simulink library "lib_AC_GFL"  (R2026a)
settings: Solver=VariableStepAuto
undefined symbols (not defined in the file): block_buses, block_idx, block_toM, buses_lf, CCVSC_idx, fref, invL, iPs_lf, iQs_lf, iTf, op_GFL
libraries: sl_discontinuities x2
settings Model: Creator=atomas  LastModifiedBy=atomas

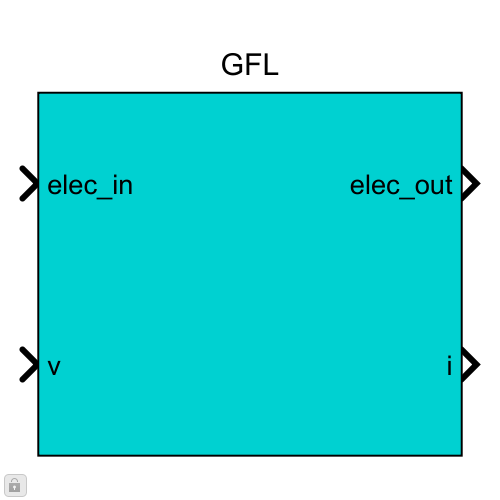
[thumbnail: Simulink's stored preview of the top-level diagram]
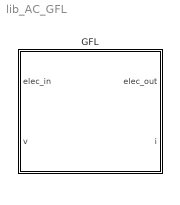
== system lib_AC_GFL ==
  GFL : Subsystem  mask(GFl){Pmax=0, Qmax=0, fb=50, dynamic_CC=Static, Tint=0.1, Kint=1, Bint=1, Lf=0.01, Rf=0.001, dynamic_PLL=Dynamic, kpi=1, kii=10, Tf=0, alphapcoef=0, alphaqcoef=0, Prel=1, Qrel=1, Eref=1}
      mask prompts: Pmax "Active power limit (p.u.)"; Qmax "Reactive power limit (p.u.)"; fb "Base frequency (Hz)"; dynamic_CC "Dynamic behaviour"; Lf "Filter inductance"; Rf "Filter resistance"; dynamic_PLL "Dynamic behaviour"; Tf "LPF time constant (s)"; alphapcoef "P droop coefficient"; alphaqcoef "Q droop coefficient"; Prel "P/P_NmP"; Qrel "Q/Q_NnQ"; Eref "Nominal voltage of PCC"
      mask help: Grid-following converter. CC is the current controller. Dynamic behavior includes the PI controller, decoupling and output inductance. Static behavior consists of setting the reference current directly in the output. PC is the power controller including the current reference calculation and low-pass filters for the power measurements.
      mask init:
      | [block_buses, block_idx, block_toM, block_fref, iTf, use_Tf, cc_mode, pll_mode] = mask_init_GFL(gcb, Tf, dynamic_CC, dynamic_PLL);
      mask Help: web('doc_GFl.html')
      mask TypeOptions dynamic_CC: Dynamic | Static
      mask TypeOptions dynamic_PLL: Dynamic | Static
      mask DialogControl CC Prompt: CC
      mask DialogControl PLL Prompt: PLL
      mask DialogControl PC Prompt: PC

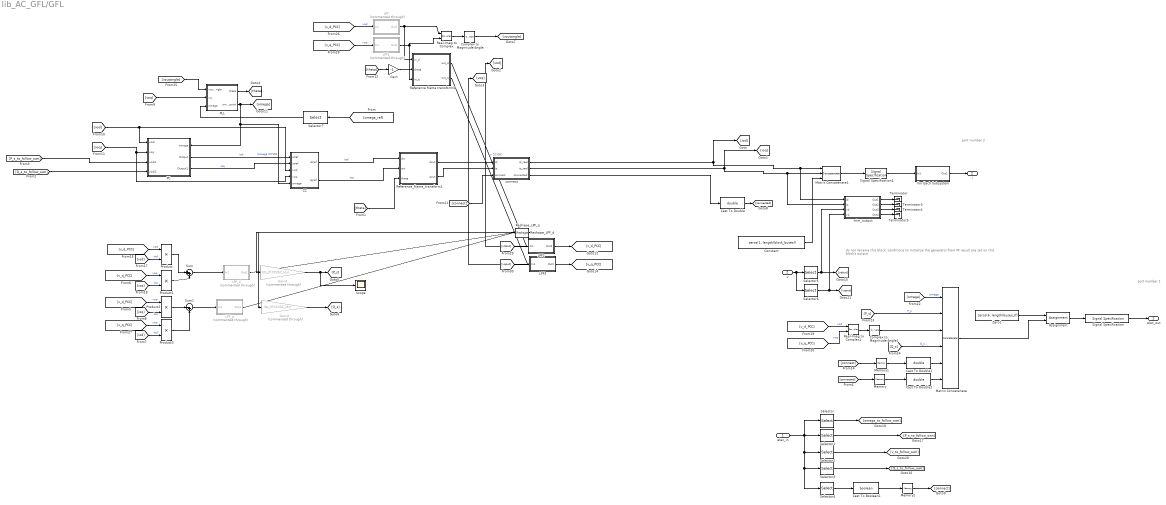
== system lib_AC_GFL/GFL ==
  note: do not rename this block, conditions to initialise the generator from PF result are set on this block's output
  note: port number 1
  note: port number 2
  elec_in : Inport
  v : Inport  Port=2
  Assignment : Assignment  NumberOfDimensions=2  DiagnosticForDimensions=Warning  IndexOptions=Assign all,Index vector (dialog)  Indices=1,block_idx  OutputSizes=1,1
  CC : Subsystem  Variant=on
  Cast To Boolean1 : DataTypeConversion  OutDataTypeStr=boolean  SaturateOnIntegerOverflow=off  RndMeth=Floor
  Cast To Double : DataTypeConversion  OutDataTypeStr=double  SaturateOnIntegerOverflow=off  RndMeth=Floor
  Cast To Double1 : DataTypeConversion  OutDataTypeStr=double  SaturateOnIntegerOverflow=off  RndMeth=Floor
  Cast To Double2 : DataTypeConversion  OutDataTypeStr=double  SaturateOnIntegerOverflow=off  RndMeth=Floor
  Complex to Magnitude-Angle : ComplexToMagnitudeAngle  Output=Angle
  Complex to Magnitude-Angle1 : ComplexToMagnitudeAngle  Output=Magnitude
  Constant : Constant  Value=zeros(1, length(block_buses))  VectorParams1D=off
  For Each Subsystem : Subsystem  TreatAsAtomicUnit=on
  Gain : Gain  Gain=-1
  Gain3 : Gain  Commented=through  Gain=iQs_lf(CCVSC_idx)
  Gain4 : Gain  Commented=through  Gain=iPs_lf(CCVSC_idx)
  LPF : Subsystem  Commented=through
  LPF1 : Subsystem  Commented=through
  LPF2 : Subsystem
  LPF3 : Subsystem
  LPF_d : Subsystem  Commented=through  Variant=on
  LPF_q : Subsystem  Commented=through  Variant=on
  Matrix Concatenate : Concatenate  NumInputs=6  Mode=Multidimensional array
  Matrix Concatenate1 : Concatenate  NumInputs=3  Mode=Multidimensional array
  Memory : Memory  InitialCondition=1
  Memory1 : Memory  InitialCondition=1
  Memory2 : Memory  InitialCondition=1
  PC : Subsystem
      settings: PortSchema="{\"entries\":[{\"content\":{\"sides\":[{\"content\":{\"connectorIds\":[\"In1\",\"In2\",\"In3\",\"In4\"]},\"type\":\"ConnectorPlacement.EquallySpacedRectSide\",\"uuid\":\"7748ce6f-2dcc-431c-b3ea-0be9c3088b1d\"},{\"content\":{\"connectorIds\":[\"In5\",\"Out1\",\"Out2\"],\"side\":\"RIGHT\"},\"type\":\"ConnectorPlacement.EquallySpacedRectSide\",\"uuid\":\"af86fd8d-043b-4d20-8ee8-e7a977d706a8\"},{\"content\":{\"connectorIds\":[],\"side\":\"TOP\"},\"type\":\"ConnectorPlacement.EquallySpacedRectSide\",\"uuid\":\"807e0dc6-0d59-4ea5-9557-3ccfd29c2ad0\"}]},\"type\":\"ConnectorPlacement.EquallySpacedConnector\",\"uuid\":\"c7fe00c5-0a0a-4038-b7ac-e659fb2aa4a7\"}],\"packageUris\":[\"http://schema.mathworks.com/mf0/Connector/R2020b\"],\"version\":\"1.0\"}"
  PLL : Subsystem  Variant=on
  Product{,1..3} (4 alike) : Product
  Real-Imag to Complex : RealImagToComplex
  Real-Imag to Complex1 : RealImagToComplex
  Reference frame transform3 : Subsystem
  Reference_frame_transform1 : Subsystem
  Reshape_LPF_d : Reshape  OutputDimensionality=Row vector (2-D)
  Reshape_LPF_q : Reshape  OutputDimensionality=Row vector (2-D)
  Scope : Scope
      settings: DataLoggingVariableName=ScopeData8
  Selector : Selector  NumberOfDimensions=2  InputPortWidth=3  IndexOptions=Index vector (dialog),Index vector (dialog)  Indices=1,block_idx  OutputSizes=1,1
  Selector1 : Selector  NumberOfDimensions=2  InputPortWidth=3  IndexOptions=Index vector (dialog),Index vector (dialog)  Indices=2,block_idx  OutputSizes=1,1
  Selector2 : Selector  NumberOfDimensions=2  InputPortWidth=3  IndexOptions=Index vector (dialog),Index vector (dialog)  Indices=3,block_idx  OutputSizes=1,1
  Selector3 : Selector  NumberOfDimensions=2  InputPortWidth=3  IndexOptions=Index vector (dialog),Index vector (dialog)  Indices=4,block_idx  OutputSizes=1,1
  Selector4 : Selector  NumberOfDimensions=2  InputPortWidth=3  IndexOptions=Index vector (dialog),Index vector (dialog)  Indices=5,block_idx  OutputSizes=1,1
  Selector5 : Selector  NumberOfDimensions=2  InputPortWidth=3  IndexOptions=Index vector (dialog),Index vector (dialog)  Indices=1,block_buses  OutputSizes=1,1
  Selector6 : Selector  NumberOfDimensions=2  InputPortWidth=3  IndexOptions=Index vector (dialog),Index vector (dialog)  Indices=2,block_buses  OutputSizes=1,1
  Selector7 : Selector  InputPortWidth=length(fref.ref_units)  IndexOptions=Index vector (dialog)  Indices=block_fref  OutputSizes=1
  Signal Specification : SignalSpecification  Dimensions=[6 length(buses_lf)]
  Signal Specification1 : SignalSpecification  Dimensions=[3 length(block_buses)]
  Sum : Sum  Inputs=|++
  Sum1 : Sum  Inputs=|-+
  Terminator{,3..5} (4 alike) : Terminator
  Zero1 : Constant  Value=zeros(6, length(buses_lf))  VectorParams1D=off  OutDataTypeStr=Inherit: Inherit via back propagation
  connect : Subsystem
  trim_output : Subsystem
  elec_out : Outport
  i : Outport  Port=2
  wires:
  Sum1/1 -> LPF_q/1(In1)
  Sum/1 -> LPF_d/1(In1)
  [voutangle] -> PLL/1(voutangle)
  [Q_s_to_follow_own] -> PC/4(vodi2)
  [P_s_to_follow_own] -> PC/3(vodi1)
  connect/3(connected) -> Cast To Double/1
  CC/2(iqiref) -> Reference_frame_transform1/2(qin)  "ioq"
  CC/1(idiref) -> Reference_frame_transform1/1(din)  "iod"
  PLL/1(theta) -> [theta]
  [omega_ref] -> Selector7/1
  [voq] -> PLL/2(vq)
  [theta] -> Reference_frame_transform1/3(theta)
  Gain/1 -> Reference frame transform3/2(theta)
  [theta] -> Gain/1
  PC/2(Output1) -> CC/2(iqref)  "ioq"
  PC/1(Output) -> CC/1(idref)  "iod"
  [v_q_PCC] -> Product3/1  "voq"
  [v_d_PCC] -> Product2/1  "vod"
  [ioq] -> Product1/2  "ioq"
  [iod] -> Product/2  "iod"
  [v_d_PCC] -> Product/1  "vod"
  Gain3/1 -> [Q_s]
  Gain4/1 -> Scope/1, [P_s]
  Product/1 -> Sum/1
  Product3/1 -> Sum1/2
  Product1/1 -> Sum/2
  Product2/1 -> Sum1/1
  [ioq] -> Product2/2  "ioq"
  [iod] -> Product3/2  "iod"
  [v_q_PCC] -> Product1/1  "voq"
  [voq] -> PC/2(voq), CC/4(voq)
  [vod] -> PC/1(vodi), CC/3(vod)
  Real-Imag to Complex/1 -> Complex to Magnitude-Angle/1
  Complex to Magnitude-Angle/1 -> [voutangle]
  PLL/2(omega_point) -> PC/5(omega), CC/5(omega), [omega]  "\\omega CCVSC"
  Reference_frame_transform1/2(qout) -> connect/2(iq)
  Reference_frame_transform1/1(dout) -> connect/1(id)
  Selector3/1 -> [Q_s_to_follow_own]
  Selector2/1 -> [v_to_follow_own]
  Selector/1 -> [omega_to_follow_own]
  [omega] -> Matrix Concatenate/1  "omega"
  [P_s] -> Matrix Concatenate/2  "P_s"
  [Q_s] -> Matrix Concatenate/4  "Q_s"
  [connected] -> Memory/1
  [connect] -> Memory1/1
  Cast To Double/1 -> [connected]
  [connect] -> connect/3(connect)
  connect/1(id_real) -> [iod], trim_output/1(id), Matrix Concatenate1/1
  connect/2(iq_real) -> [ioq], trim_output/2(iq), Matrix Concatenate1/2
  [v_d_PCC] -> Real-Imag to Complex1/1  "vod"
  [v_q_PCC] -> Real-Imag to Complex1/2  "voq"
  Real-Imag to Complex1/1 -> Complex to Magnitude-Angle1/1
  Complex to Magnitude-Angle1/1 -> Matrix Concatenate/3
  [v_d_PCC] -> LPF/1(In1)  "vod"
  [v_q_PCC] -> LPF1/1(In1)  "voq"
  Selector4/1 -> Cast To Boolean1/1
  Cast To Boolean1/1 -> Memory2/1
  Cast To Double1/1 -> Matrix Concatenate/5
  Cast To Double2/1 -> Matrix Concatenate/6
  Zero1/1 -> Assignment/1
  Signal Specification/1 -> elec_out/1
  Assignment/1 -> Signal Specification/1
  Matrix Concatenate/1 -> Assignment/2
  elec_in/1 -> Selector4/1, Selector3/1, Selector2/1, Selector1/1, Selector/1
  Matrix Concatenate1/1 -> Signal Specification1/1
  Signal Specification1/1 -> For Each Subsystem/1(In1)
  Constant/1 -> Matrix Concatenate1/3
  For Each Subsystem/1(Out1) -> i/1
  trim_output/1(Out1) -> Terminator/1
  trim_output/3(Out3) -> Terminator4/1
  trim_output/2(Out2) -> Terminator3/1
  trim_output/4(Out4) -> Terminator5/1
  Selector5/1 -> trim_output/3(vd), [vdout]
  Selector6/1 -> trim_output/4(vq), [vqout]
  v/1 -> Selector6/1, Selector5/1
  Memory/1 -> Cast To Double2/1
  Selector1/1 -> [P_s_to_follow_own]
  Memory1/1 -> Cast To Double1/1
  Memory2/1 -> [connect]
  LPF/1(Out1) -> Reference frame transform3/1(in_d), Real-Imag to Complex/1
  LPF1/1(Out1) -> Real-Imag to Complex/2, Reference frame transform3/3(in_q)
  Selector7/1 -> PLL/3(omega)
  [vdout] -> [v_d_PCC]
  [vqout] -> [v_q_PCC]
  Reference frame transform3/1(out_d) -> LPF2/1(In1)  "v CCVSC"
  LPF2/1(Out1) -> [vod]
  Reference frame transform3/2(out_q) -> LPF3/1(In1)
  LPF3/1(Out1) -> [voq]
  LPF_d/1(Out1) -> Reshape_LPF_d/1
  Reshape_LPF_d/1 -> Gain4/1
  LPF_q/1(Out1) -> Reshape_LPF_q/1
  Reshape_LPF_q/1 -> Gain3/1

== system lib_AC_GFL/GFL/CC ==
  note: 1) Add Subsystem or Model blocks as valid variant choices.
      | 2) You cannot connect blocks at this level. At simulation, connectivity is automatically
      | determined, based on the active variant and port name matching.
  idref : Inport
  iqref : Inport  Port=2
  vod : Inport  Port=3
  voq : Inport  Port=4
  omega : Inport  Port=5
  dynamic : Subsystem  VariantControl=cc_mode == 1  mask{dynamic_line=Dynamic}
      mask prompts: dynamic_line "Line"
      mask TypeOptions dynamic_line: RL/dynamic
  static : Subsystem  VariantControl=(default)
  idiref : Outport
  iqiref : Outport  Port=2

== system lib_AC_GFL/GFL/For Each Subsystem ==
  In1 : Inport  Partition=on  PartitionDimension=1  PartitionWidth=1  PartitionOffset=0
  For Each : ForEach  DisableCoverage=on
  State-Space : StateSpace  A=[]  B=[]  C=[]  D=block_toM  InitialCondition=0  ParameterTunability=Optimized
  Transpose : Math  Operator=transpose
  Transpose1 : Math  Operator=transpose
  Out1 : Outport  ConcatenationDimension=1
  wires:
  Transpose1/1 -> Out1/1
  In1/1 -> Transpose/1
  Transpose/1 -> State-Space/1
  State-Space/1 -> Transpose1/1

== system lib_AC_GFL/GFL/LPF ==
  In1 : Inport
  Gain : Gain  Gain=1e2
  I : Integrator  InitialCondition=op_GFL.LPF_I
  Sum4 : Sum  Inputs=|+-
  Out1 : Outport
  wires:
  Gain/1 -> I/1
  Sum4/1 -> Gain/1
  In1/1 -> Sum4/1
  I/1 -> Out1/1, Sum4/2

== system lib_AC_GFL/GFL/LPF1 ==
  In1 : Inport
  Gain : Gain  Gain=1e2
  I : Integrator  InitialCondition=op_GFL.LPF1_I
  Sum4 : Sum  Inputs=|+-
  Out1 : Outport
  wires:
  I/1 -> Sum4/2, Out1/1
  In1/1 -> Sum4/1
  Sum4/1 -> Gain/1
  Gain/1 -> I/1

== system lib_AC_GFL/GFL/LPF2 ==
  In1 : Inport
  Gain : Gain  Gain=1e2
  I : Integrator  InitialCondition=op_GFL.LPF2_I
  Sum4 : Sum  Inputs=|+-
  Out1 : Outport
  wires:
  Gain/1 -> I/1
  Sum4/1 -> Gain/1
  In1/1 -> Sum4/1
  I/1 -> Out1/1, Sum4/2

== system lib_AC_GFL/GFL/LPF3 ==
  In1 : Inport
  Gain : Gain  Gain=1e2
  I : Integrator  InitialCondition=op_GFL.LPF3_I
  Sum4 : Sum  Inputs=|+-
  Out1 : Outport
  wires:
  I/1 -> Sum4/2, Out1/1
  In1/1 -> Sum4/1
  Sum4/1 -> Gain/1
  Gain/1 -> I/1

== system lib_AC_GFL/GFL/LPF_d ==
  note: 1) Add Subsystem or Model blocks as valid variant choices.
      | 2) You cannot connect blocks at this level. At simulation, connectivity is automatically
      | determined, based on the active variant and port name matching.
  In1 : Inport
  Active : Subsystem  VariantControl=use_Tf == 1
  Bypass : Subsystem  VariantControl=(default)
  Out1 : Outport

== system lib_AC_GFL/GFL/LPF_q ==
  note: 1) Add Subsystem or Model blocks as valid variant choices.
      | 2) You cannot connect blocks at this level. At simulation, connectivity is automatically
      | determined, based on the active variant and port name matching.
  In1 : Inport
  Active : Subsystem  VariantControl=use_Tf == 1
  Bypass : Subsystem  VariantControl=(default)
  Out1 : Outport

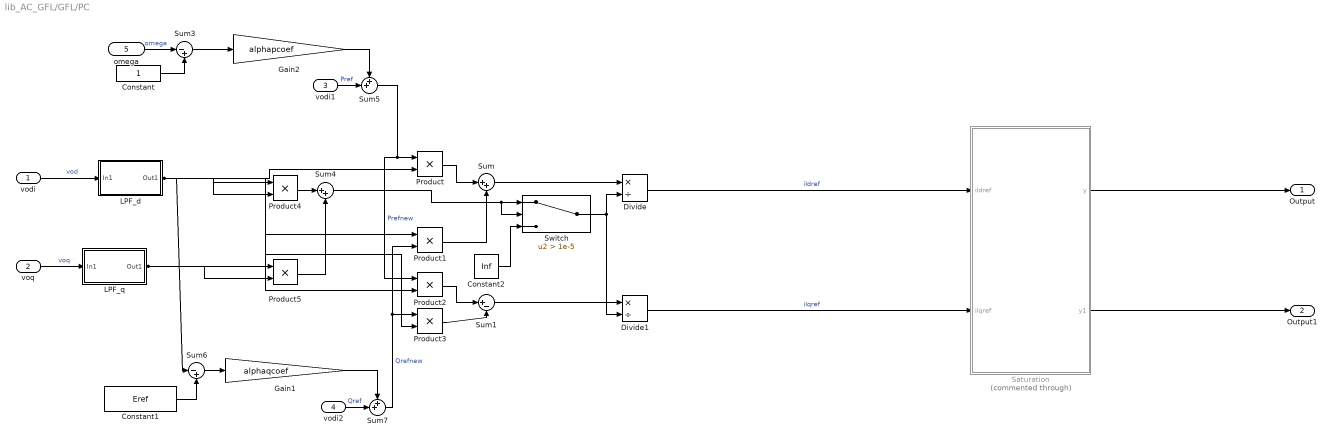
== system lib_AC_GFL/GFL/PC ==
  vodi : Inport
  voq : Inport  Port=2
  vodi1 : Inport  Port=3
  vodi2 : Inport  Port=4
  omega : Inport  Port=5
  Constant : Constant
  Constant1 : Constant  Value=Eref  VectorParams1D=off
  Constant2 : Constant  Value=Inf
  Divide : Product  Inputs=*/
  Divide1 : Product  Inputs=*/
  Gain1 : Gain  Gain=alphaqcoef
  Gain2 : Gain  Gain=alphapcoef
  LPF_d : Subsystem  Variant=on
  LPF_q : Subsystem  Variant=on
  Product{,1..5} (6 alike) : Product
  Saturation : Subsystem  Commented=through
  Sum : Sum  Inputs=|++
  Sum1 : Sum  Inputs=|+-
  Sum3 : Sum  Inputs=|-+
  Sum4 : Sum  Inputs=|++
  Sum5 : Sum  Inputs=++|
  Sum6 : Sum  Inputs=|-+
  Sum7 : Sum  Inputs=++|
  Switch : Switch  Criteria=u2 > Threshold  Threshold=1e-5  ZeroCross=off  SaturateOnIntegerOverflow=off  InputSameDT=off
  Output : Outport
  Output1 : Outport  Port=2
  wires:
  LPF_q/1(Out1) -> Product5/1, Product5/2, Product2/2, Product1/1
  voq/1 -> LPF_q/1(In1)  "voq"
  LPF_d/1(Out1) -> Product4/1, Product4/2, Product/2, Product3/2, Sum6/1
  vodi/1 -> LPF_d/1(In1)  "vod"
  Switch/1 -> Divide1/2, Divide/2
  Constant2/1 -> Switch/3
  vodi2/1 -> Sum7/2  "Qref"
  Sum6/1 -> Gain1/1
  omega/1 -> Sum3/1  "omega"
  Gain1/1 -> Sum7/1
  Constant1/1 -> Sum6/2
  vodi1/1 -> Sum5/2  "Pref"
  Gain2/1 -> Sum5/1
  Constant/1 -> Sum3/2
  Sum3/1 -> Gain2/1
  Sum/1 -> Divide/1
  Sum4/1 -> Switch/1, Switch/2
  Sum1/1 -> Divide1/1
  Sum5/1 -> Product/1, Product2/1  "Prefnew"
  Product5/1 -> Sum4/2
  Product4/1 -> Sum4/1
  Sum7/1 -> Product3/1, Product1/2  "Qrefnew"
  Product3/1 -> Sum1/2
  Product2/1 -> Sum1/1
  Product1/1 -> Sum/2
  Product/1 -> Sum/1
  Divide/1 -> Saturation/1(ildref)  "ildref"
  Divide1/1 -> Saturation/2(ilqref)  "ilqref"
  Saturation/1(y) -> Output/1
  Saturation/2(y1) -> Output1/1

== system lib_AC_GFL/GFL/PLL ==
  note: 1) Add Subsystem or Model blocks as valid variant choices.
      | 2) You cannot connect blocks at this level. At simulation, connectivity is automatically
      | determined, based on the active variant and port name matching.
  voutangle : Inport
  vq : Inport  Port=2
  omega : Inport  Port=3
  dynamic : Subsystem  VariantControl=pll_mode == 1
  static : Subsystem  VariantControl=(default)
  theta : Outport
  omega_point : Outport  Port=2

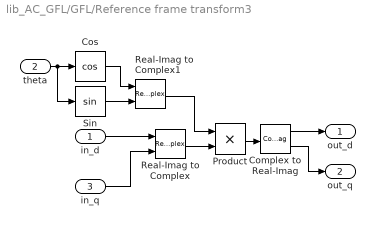
== system lib_AC_GFL/GFL/Reference frame transform3 ==
  in_d : Inport
  theta : Inport  Port=2
  in_q : Inport  Port=3
  Complex to Real-Imag : ComplexToRealImag
  Cos : Trigonometry  SCDEnableBlockLinearizationSpecification=on  Operator=cos
  Product : Product
  Real-Imag to Complex : RealImagToComplex
  Real-Imag to Complex1 : RealImagToComplex
  Sin : Trigonometry  SCDEnableBlockLinearizationSpecification=on
  out_d : Outport
  out_q : Outport  Port=2
  wires:
  Complex to Real-Imag/2 -> out_q/1
  Real-Imag to Complex1/1 -> Product/1
  Real-Imag to Complex/1 -> Product/2
  Product/1 -> Complex to Real-Imag/1
  theta/1 -> Sin/1, Cos/1
  Cos/1 -> Real-Imag to Complex1/1
  Sin/1 -> Real-Imag to Complex1/2
  Complex to Real-Imag/1 -> out_d/1
  in_q/1 -> Real-Imag to Complex/2
  in_d/1 -> Real-Imag to Complex/1

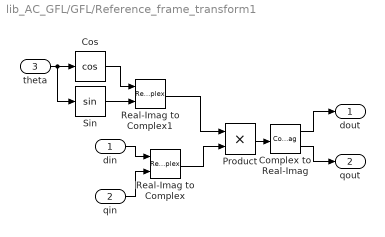
== system lib_AC_GFL/GFL/Reference_frame_transform1 ==
  din : Inport
  qin : Inport  Port=2
  theta : Inport  Port=3
  Complex to Real-Imag : ComplexToRealImag
  Cos : Trigonometry  SCDEnableBlockLinearizationSpecification=on  Operator=cos
  Product : Product
  Real-Imag to Complex : RealImagToComplex
  Real-Imag to Complex1 : RealImagToComplex
  Sin : Trigonometry  SCDEnableBlockLinearizationSpecification=on
  dout : Outport
  qout : Outport  Port=2
  wires:
  Sin/1 -> Real-Imag to Complex1/2
  Cos/1 -> Real-Imag to Complex1/1
  theta/1 -> Cos/1, Sin/1
  Product/1 -> Complex to Real-Imag/1
  Real-Imag to Complex/1 -> Product/2
  qin/1 -> Real-Imag to Complex/2
  din/1 -> Real-Imag to Complex/1
  Real-Imag to Complex1/1 -> Product/1
  Complex to Real-Imag/2 -> qout/1
  Complex to Real-Imag/1 -> dout/1

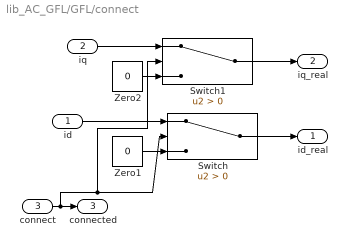
== system lib_AC_GFL/GFL/connect ==
  id : Inport
  iq : Inport  Port=2
  connect : Inport  Port=3
  Switch : Switch  Criteria=u2 > Threshold  ZeroCross=off  SaturateOnIntegerOverflow=off  InputSameDT=off
  Switch1 : Switch  Criteria=u2 > Threshold  ZeroCross=off  SaturateOnIntegerOverflow=off  InputSameDT=off
  Zero1 : Constant  Value=0  VectorParams1D=off  OutDataTypeStr=Inherit: Inherit via back propagation
  Zero2 : Constant  Value=0  VectorParams1D=off  OutDataTypeStr=Inherit: Inherit via back propagation
  id_real : Outport
  iq_real : Outport  Port=2
  connected : Outport  Port=3  OutDataTypeStr=boolean
  wires:
  Switch/1 -> id_real/1
  Zero1/1 -> Switch/3
  id/1 -> Switch/1
  connect/1 -> connected/1, Switch1/2, Switch/2
  Switch1/1 -> iq_real/1
  iq/1 -> Switch1/1
  Zero2/1 -> Switch1/3

== system lib_AC_GFL/GFL/trim_output ==
  id : Inport
  iq : Inport  Port=2
  vd : Inport  Port=3
  vq : Inport  Port=4
  Out1 : Outport
  Out2 : Outport  Port=2
  Out3 : Outport  Port=3
  Out4 : Outport  Port=4
  wires:
  id/1 -> Out1/1
  vq/1 -> Out4/1
  vd/1 -> Out3/1
  iq/1 -> Out2/1

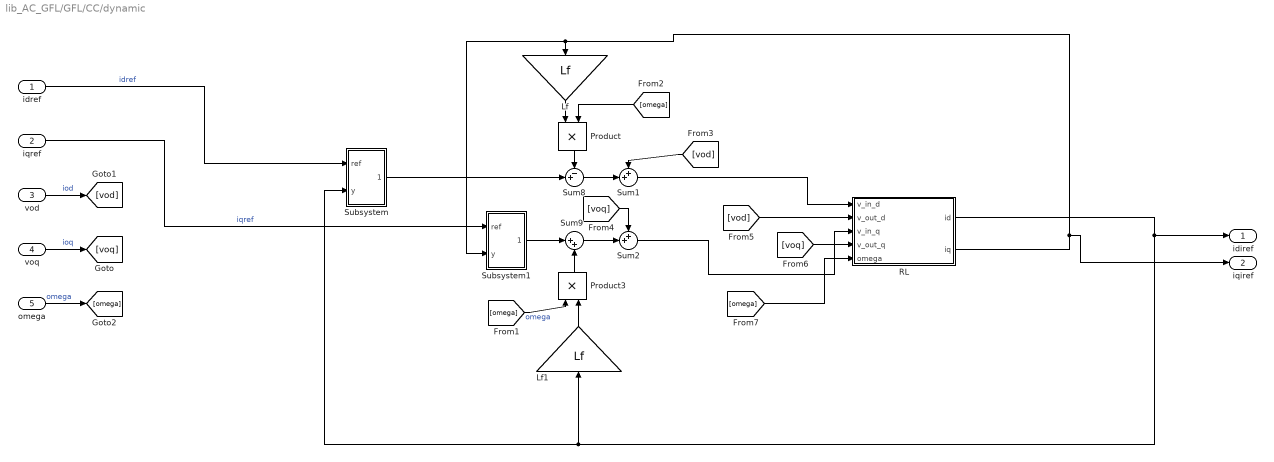
== system lib_AC_GFL/GFL/CC/dynamic ==
  idref : Inport
  iqref : Inport  Port=2
  vod : Inport  Port=3
  voq : Inport  Port=4
  omega : Inport  Port=5
  "Lf " : Gain  Gain=Lf
  Lf1 : Gain  Gain=Lf
  Product : Product
  Product3 : Product
  RL : Subsystem  Variant=on  mask(Line){dynamic=Dynamic, R=Rf, L=Lf}
      mask prompts: dynamic "Dynamic behavior"; R "Series resistance (p.u.)"; L "Inductance (p.u.)"
      mask init:
      | [invL, omegab, rl_mode] = mask_init_RL(dynamic, L, 50);
      mask Help: web('Documentation/RL.html')
      mask TypeOptions dynamic: Static | Dynamic | Static omega
  Subsystem : Subsystem
  Subsystem1 : Subsystem
  Sum1 : Sum  Inputs=++|
  Sum2 : Sum  Inputs=++|
  Sum8 : Sum  Inputs=-+|
  Sum9 : Sum  Inputs=|++
  idiref : Outport
  iqiref : Outport  Port=2
  wires:
  RL/2(iq) -> iqiref/1, Subsystem1/2(y), "Lf "/1
  Subsystem1/1(Out1) -> Sum9/1
  [omega] -> Product3/1  "omega"
  "Lf "/1 -> Product/1
  Product3/1 -> Sum9/2
  Lf1/1 -> Product3/2
  [omega] -> Product/2
  Product/1 -> Sum8/1
  iqref/1 -> Subsystem1/1(ref)  "iqref"
  Sum8/1 -> Sum1/2
  Sum9/1 -> Sum2/2
  [vod] -> Sum1/1
  [voq] -> Sum2/1
  omega/1 -> [omega]  "omega"
  voq/1 -> [voq]  "ioq"
  vod/1 -> [vod]  "iod"
  [vod] -> RL/2(v_out_d)
  [voq] -> RL/4(v_out_q)
  Sum1/1 -> RL/1(v_in_d)
  Sum2/1 -> RL/3(v_in_q)
  RL/1(id) -> Subsystem/2(y), Lf1/1, idiref/1
  idref/1 -> Subsystem/1(ref)  "idref"
  Subsystem/1(Out1) -> Sum8/2
  [omega] -> RL/5(omega)

== system lib_AC_GFL/GFL/CC/static ==
  idref : Inport
  iqref : Inport  Port=2
  vod : Inport  Port=3
  voq : Inport  Port=4
  omega : Inport  Port=5
  Terminator : Terminator
  Terminator1 : Terminator
  Terminator2 : Terminator
  idiref : Outport
  iqiref : Outport  Port=2
  wires:
  voq/1 -> Terminator1/1  "voq"
  vod/1 -> Terminator/1  "vod"
  idref/1 -> idiref/1  "idref"
  iqref/1 -> iqiref/1  "iqref"
  omega/1 -> Terminator2/1  "omega"

== system lib_AC_GFL/GFL/LPF_d/Active ==
  In1 : Inport
  Impl : Subsystem
  Out1 : Outport
  wires:
  Impl/1(Out1) -> Out1/1
  In1/1 -> Impl/1(In1)

== system lib_AC_GFL/GFL/LPF_d/Bypass ==
  In1 : Inport
  Reshape_row : Reshape  OutputDimensionality=Row vector (2-D)
  Out1 : Outport
  wires:
  In1/1 -> Reshape_row/1
  Reshape_row/1 -> Out1/1

== system lib_AC_GFL/GFL/LPF_q/Active ==
  In1 : Inport
  Impl : Subsystem
  Out1 : Outport
  wires:
  Impl/1(Out1) -> Out1/1
  In1/1 -> Impl/1(In1)

== system lib_AC_GFL/GFL/LPF_q/Bypass ==
  In1 : Inport
  Reshape_row : Reshape  OutputDimensionality=Row vector (2-D)
  Out1 : Outport
  wires:
  In1/1 -> Reshape_row/1
  Reshape_row/1 -> Out1/1

== system lib_AC_GFL/GFL/PC/LPF_d ==
  note: 1) Add Subsystem or Model blocks as valid variant choices.
      | 2) You cannot connect blocks at this level. At simulation, connectivity is automatically
      | determined, based on the active variant and port name matching.
  In1 : Inport
  Active : Subsystem  VariantControl=use_Tf == 1
  Bypass : Subsystem  VariantControl=(default)
  Out1 : Outport

== system lib_AC_GFL/GFL/PC/LPF_q ==
  note: 1) Add Subsystem or Model blocks as valid variant choices.
      | 2) You cannot connect blocks at this level. At simulation, connectivity is automatically
      | determined, based on the active variant and port name matching.
  In1 : Inport
  Active : Subsystem  VariantControl=use_Tf == 1
  Bypass : Subsystem  VariantControl=(default)
  Out1 : Outport

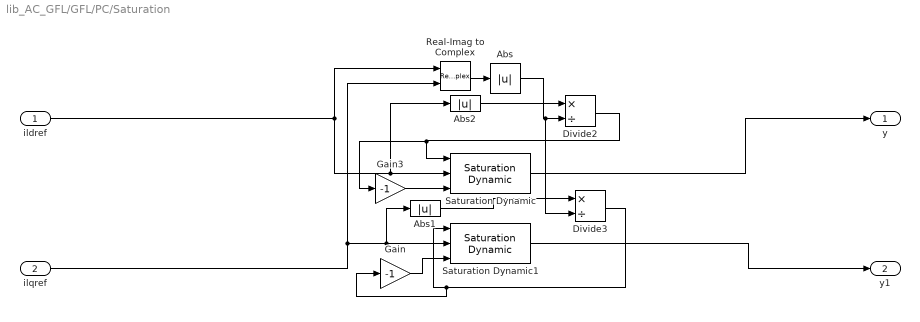
== system lib_AC_GFL/GFL/PC/Saturation ==
  ildref : Inport
  ilqref : Inport  Port=2
  Abs : Abs  ZeroCross=off  SaturateOnIntegerOverflow=off
  Abs1 : Abs  ZeroCross=off  SaturateOnIntegerOverflow=off
  Abs2 : Abs  ZeroCross=off  SaturateOnIntegerOverflow=off
  Divide2 : Product  Inputs=*/
  Divide3 : Product  Inputs=*/
  Gain : Gain  Gain=-1
  Gain3 : Gain  Gain=-1
  Real-Imag to Complex : RealImagToComplex
  Saturation Dynamic : sl_discontinuities/Saturation Dynamic  OutMin=[]  OutMax=[]  OutDataTypeStr=Inherit: Same as second input  OutDataType=fixdt(1, 16)  OutScaling=2^-10  DoSatur=off
  Saturation Dynamic1 : sl_discontinuities/Saturation Dynamic  OutMin=[]  OutMax=[]  OutDataTypeStr=Inherit: Same as second input  OutDataType=fixdt(1, 16)  OutScaling=2^-10  DoSatur=off
  y : Outport
  y1 : Outport  Port=2
  wires:
  Gain/1 -> Saturation Dynamic1/3
  Divide3/1 -> Gain/1, Saturation Dynamic1/1
  Divide2/1 -> Gain3/1, Saturation Dynamic/1
  Saturation Dynamic/1 -> y/1
  Abs/1 -> Divide3/2, Divide2/2
  Gain3/1 -> Saturation Dynamic/3
  Abs1/1 -> Divide3/1
  Real-Imag to Complex/1 -> Abs/1
  ilqref/1 -> Abs1/1, Saturation Dynamic1/2, Real-Imag to Complex/2
  Abs2/1 -> Divide2/1
  ildref/1 -> Abs2/1, Saturation Dynamic/2, Real-Imag to Complex/1
  Saturation Dynamic1/1 -> y1/1

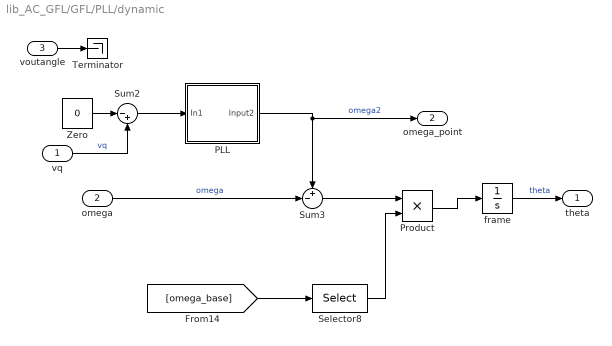
== system lib_AC_GFL/GFL/PLL/dynamic ==
  vq : Inport
  omega : Inport  Port=2
  voutangle : Inport  Port=3
  PLL : Subsystem
  Product : Product
  Selector8 : Selector  InputPortWidth=length(fref.ref_units)  IndexOptions=Index vector (dialog)  Indices=block_fref  OutputSizes=1
  Sum2 : Sum  Inputs=|-+
  Sum3 : Sum  Inputs=+-|
  Terminator : Terminator
  Zero : Constant  Value=0  OutDataTypeStr=Inherit: Inherit via back propagation
  frame : Integrator  InitialCondition=op_GFL.PLL_dynamic_frame  UpperSaturationLimit=pi  LowerSaturationLimit=-pi
  theta : Outport
  omega_point : Outport  Port=2
  wires:
  voutangle/1 -> Terminator/1
  vq/1 -> Sum2/2  "vq"
  omega/1 -> Sum3/2  "omega"
  Zero/1 -> Sum2/1
  frame/1 -> theta/1  "theta"
  Product/1 -> frame/1
  PLL/1(Input2) -> omega_point/1, Sum3/1  "omega2"
  Sum3/1 -> Product/1
  Sum2/1 -> PLL/1(In1)
  [omega_base] -> Selector8/1
  Selector8/1 -> Product/2

== system lib_AC_GFL/GFL/PLL/static ==
  vq : Inport
  omega : Inport  Port=2
  voutangle : Inport  Port=3
  Gain : Gain  Gain=-1
  IC : InitialCondition  Value=op_GFL.PLL_dynamic_frame
  Terminator : Terminator
  Terminator1 : Terminator
  theta : Outport
  omega_point : Outport  Port=2
  wires:
  vq/1 -> Terminator/1  "vq"
  omega/1 -> omega_point/1, Terminator1/1  "vq"
  voutangle/1 -> Gain/1
  Gain/1 -> IC/1
  IC/1 -> theta/1

== system lib_AC_GFL/GFL/CC/dynamic/RL ==
  note: 1) Add Subsystem or Model blocks as valid variant choices.
      | 2) You cannot connect blocks at this level. At simulation, connectivity is automatically
      | determined, based on the active variant and port name matching.
  v_in_d : Inport
  v_out_d : Inport  Port=2
  v_in_q : Inport  Port=3
  v_out_q : Inport  Port=4
  omega : Inport  Port=5
  dynamic : Subsystem  VariantControl=rl_mode == 1
      settings: PortSchema="{\"entries\":[{\"content\":{\"sides\":[{\"content\":{\"connectorIds\":[\"In1\"]},\"type\":\"ConnectorPlacement.EquallySpacedRectSide\",\"uuid\":\"63966e24-f9e7-4b2d-b456-7f4ea5e3f230\"},{\"content\":{\"connectorIds\":[\"In2\",\"In3\",\"In4\",\"In5\",\"Out1\",\"Out2\"],\"side\":\"RIGHT\"},\"type\":\"ConnectorPlacement.EquallySpacedRectSide\",\"uuid\":\"ded6ef04-52fd-47df-8e49-cf16b827098d\"},{\"content\":{\"side\":\"TOP\"},\"type\":\"ConnectorPlacement.EquallySpacedRectSide\",\"uuid\":\"f940a985-fa23-4968-ad44-1d76d0e20c6a\"}]},\"type\":\"ConnectorPlacement.EquallySpacedConnector\",\"uuid\":\"20f61d3c-9af2-4982-98ea-af4910e61c9c\"}],\"packageUris\":[\"http://schema.mathworks.com/mf0/Connector/R2020b\"],\"version\":\"1.0\"}"
  static : Subsystem  VariantControl=rl_mode == 2
  static_omega : Subsystem  VariantControl=(default)
  id : Outport
  iq : Outport  Port=2

== system lib_AC_GFL/GFL/CC/dynamic/Subsystem ==
  ref : Inport
  y : Inport  Port=2
  Gain : Gain  Gain=Bint
  Gain1 : Gain  Gain=1./Tint
  Gain2 : Gain  Gain=Kint
  Integrator : Integrator  InitialCondition=op_GFL.CC_dynamic_Subsystem_Integrator
  Sum : Sum  Inputs=++|
  Sum1 : Sum  Inputs=|+-
  Sum6 : Sum  Inputs=|+-
  Out1 : Outport
  wires:
  y/1 -> Sum1/2, Sum6/2
  ref/1 -> Gain/1, Sum6/1
  Gain/1 -> Sum1/1
  Sum/1 -> Gain2/1
  Sum1/1 -> Sum/1
  Sum6/1 -> Gain1/1
  Gain1/1 -> Integrator/1
  Integrator/1 -> Sum/2
  Gain2/1 -> Out1/1

== system lib_AC_GFL/GFL/CC/dynamic/Subsystem1 ==
  ref : Inport
  y : Inport  Port=2
  Gain : Gain  Gain=Bint
  Gain1 : Gain  Gain=1./Tint
  Gain2 : Gain  Gain=Kint
  Integrator : Integrator  InitialCondition=op_GFL.CC_dynamic_Subsystem1_Integrator
  Sum : Sum  Inputs=++|
  Sum1 : Sum  Inputs=|+-
  Sum6 : Sum  Inputs=|+-
  Out1 : Outport
  wires:
  Gain2/1 -> Out1/1
  Integrator/1 -> Sum/2
  Gain1/1 -> Integrator/1
  Sum6/1 -> Gain1/1
  Sum1/1 -> Sum/1
  Sum/1 -> Gain2/1
  Gain/1 -> Sum1/1
  ref/1 -> Sum6/1, Gain/1
  y/1 -> Sum6/2, Sum1/2

== system lib_AC_GFL/GFL/LPF_d/Active/Impl ==
  In1 : Inport
  Gain : Gain  Gain=iTf
  I : Integrator  InitialCondition=op_GFL.LPF_d_Active_Impl_I
  Sum4 : Sum  Inputs=|+-
  Out1 : Outport
  wires:
  Gain/1 -> I/1
  Sum4/1 -> Gain/1
  In1/1 -> Sum4/1
  I/1 -> Out1/1, Sum4/2

== system lib_AC_GFL/GFL/LPF_q/Active/Impl ==
  In1 : Inport
  Gain : Gain  Gain=iTf
  I : Integrator  InitialCondition=op_GFL.LPF_q_Active_Impl_I
  Sum4 : Sum  Inputs=|+-
  Out1 : Outport
  wires:
  Gain/1 -> I/1
  I/1 -> Out1/1, Sum4/2
  In1/1 -> Sum4/1
  Sum4/1 -> Gain/1

== system lib_AC_GFL/GFL/PC/LPF_d/Active ==
  In1 : Inport
  Impl : Subsystem
  Out1 : Outport
  wires:
  Impl/1(Out1) -> Out1/1
  In1/1 -> Impl/1(In1)

== system lib_AC_GFL/GFL/PC/LPF_d/Bypass ==
  In1 : Inport
  Out1 : Outport
  wires:
  In1/1 -> Out1/1

== system lib_AC_GFL/GFL/PC/LPF_q/Active ==
  In1 : Inport
  Impl : Subsystem
  Out1 : Outport
  wires:
  Impl/1(Out1) -> Out1/1
  In1/1 -> Impl/1(In1)

== system lib_AC_GFL/GFL/PC/LPF_q/Bypass ==
  In1 : Inport
  Out1 : Outport
  wires:
  In1/1 -> Out1/1

== system lib_AC_GFL/GFL/PLL/dynamic/PLL ==
  In1 : Inport
  Gain : Gain  Gain=kpi
  Gain1 : Gain  Gain=kii
  I : Integrator  InitialCondition=op_GFL.PLL_dynamic_PLL_I
  Sum10 : Sum  Inputs=|++
  Input2 : Outport
  wires:
  I/1 -> Sum10/2
  Gain/1 -> Sum10/1
  Gain1/1 -> I/1
  In1/1 -> Gain/1, Gain1/1
  Sum10/1 -> Input2/1

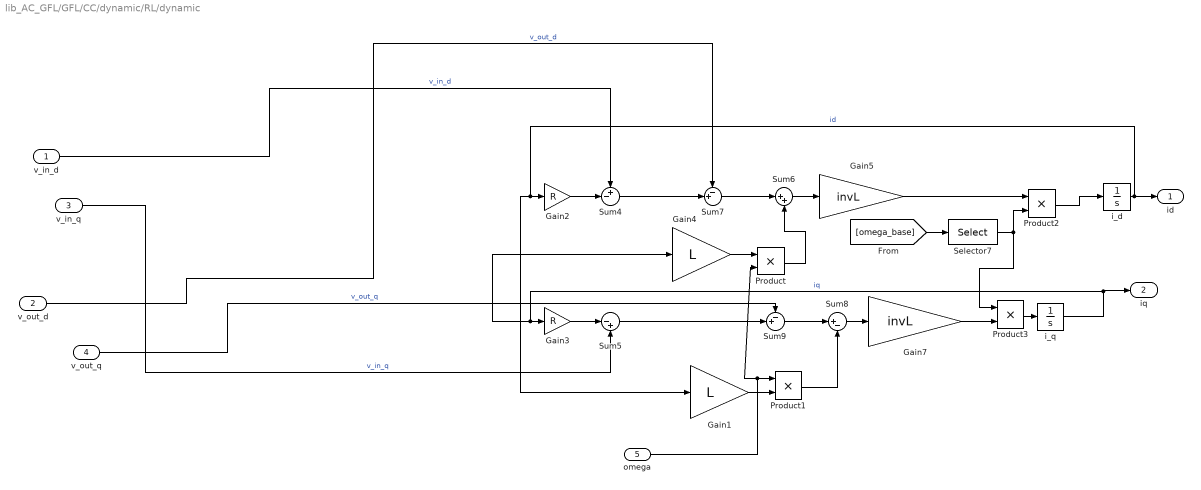
== system lib_AC_GFL/GFL/CC/dynamic/RL/dynamic ==
  v_in_d : Inport
  v_out_d : Inport  Port=2
  v_in_q : Inport  Port=3
  v_out_q : Inport  Port=4
  omega : Inport  Port=5
  Gain1 : Gain  Gain=L
  Gain2 : Gain  Gain=R
  Gain3 : Gain  Gain=R
  Gain4 : Gain  Gain=L
  Gain5 : Gain  Gain=invL
  Gain7 : Gain  Gain=invL
  Product{,1..3} (4 alike) : Product
  Selector7 : Selector  InputPortWidth=length(fref.ref_units)  IndexOptions=Index vector (dialog)  Indices=block_fref  OutputSizes=1
  Sum4 : Sum  Inputs=+-|
  Sum5 : Sum  Inputs=|-+
  Sum6 : Sum  Inputs=|++
  Sum7 : Sum  Inputs=-+|
  Sum8 : Sum  Inputs=|+-
  Sum9 : Sum  Inputs=-+|
  i_d : Integrator  InitialCondition=op_GFL.CC_dynamic_RL_dynamic_i_d
  i_q : Integrator  InitialCondition=op_GFL.CC_dynamic_RL_dynamic_i_q
  id : Outport
  iq : Outport  Port=2
  wires:
  v_out_q/1 -> Sum9/1  "v_out_q"
  v_out_d/1 -> Sum7/1  "v_out_d"
  Sum9/1 -> Sum8/1
  Gain1/1 -> Product1/2
  i_q/1 -> iq/1, Gain4/1, Gain3/1  "iq"
  Gain7/1 -> Product3/2
  Sum5/1 -> Sum9/2
  Gain3/1 -> Sum5/1
  Sum7/1 -> Sum6/1
  Gain4/1 -> Product/1
  Product1/1 -> Sum8/2
  Sum4/1 -> Sum7/2
  Sum8/1 -> Gain7/1
  Product/1 -> Sum6/2
  Sum6/1 -> Gain5/1
  i_d/1 -> id/1, Gain1/1, Gain2/1  "id"
  Gain2/1 -> Sum4/2
  v_in_d/1 -> Sum4/1  "v_in_d"
  v_in_q/1 -> Sum5/2  "v_in_q"
  omega/1 -> Product/2, Product1/1
  Gain5/1 -> Product2/1
  Product2/1 -> i_d/1
  Selector7/1 -> Product2/2, Product3/1
  [omega_base] -> Selector7/1
  Product3/1 -> i_q/1

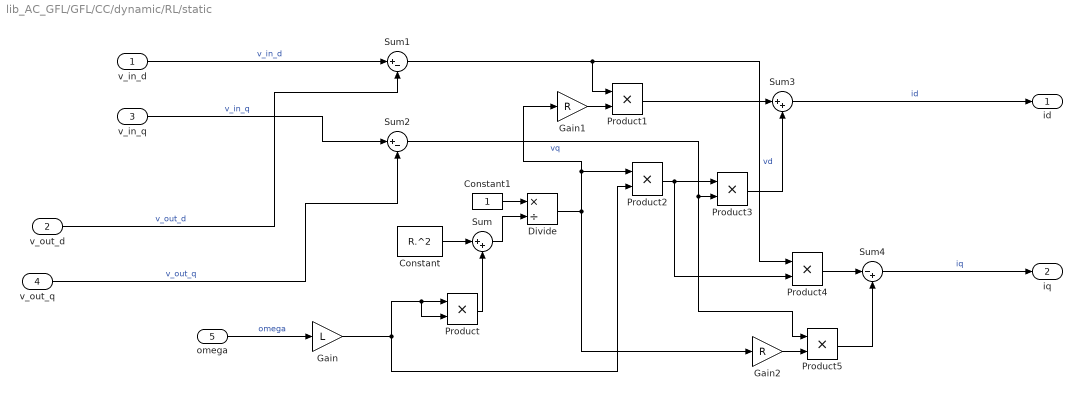
== system lib_AC_GFL/GFL/CC/dynamic/RL/static ==
  v_in_d : Inport
  v_out_d : Inport  Port=2
  v_in_q : Inport  Port=3
  v_out_q : Inport  Port=4
  omega : Inport  Port=5
  Constant : Constant  Value=R.^2
  Constant1 : Constant
  Divide : Product  Inputs=*/
  Gain : Gain  Gain=L
  Gain1 : Gain  Gain=R
  Gain2 : Gain  Gain=R
  Product{,1..5} (6 alike) : Product
  Sum : Sum  Inputs=|++
  Sum1 : Sum  Inputs=|+-
  Sum2 : Sum  Inputs=|+-
  Sum3 : Sum  Inputs=|++
  Sum4 : Sum  Inputs=|-+
  id : Outport
  iq : Outport  Port=2
  wires:
  omega/1 -> Gain/1  "omega"
  v_in_d/1 -> Sum1/1  "v_in_d"
  v_out_q/1 -> Sum2/2  "v_out_q"
  Sum4/1 -> iq/1  "iq"
  Sum3/1 -> id/1  "id"
  Gain1/1 -> Product1/2
  Product2/1 -> Product4/2, Product3/1
  Product4/1 -> Sum4/1
  Divide/1 -> Gain2/1, Gain1/1, Product2/1
  Sum1/1 -> Product1/1, Product4/1  "vd"
  Product3/1 -> Sum3/2
  Constant1/1 -> Divide/1
  Gain/1 -> Product/2, Product/1, Product2/2
  Sum2/1 -> Product5/1, Product3/2  "vq"
  Constant/1 -> Sum/1
  Product5/1 -> Sum4/2
  Product1/1 -> Sum3/1
  Product/1 -> Sum/2
  Gain2/1 -> Product5/2
  Sum/1 -> Divide/2
  v_out_d/1 -> Sum1/2  "v_out_d"
  v_in_q/1 -> Sum2/1  "v_in_q"

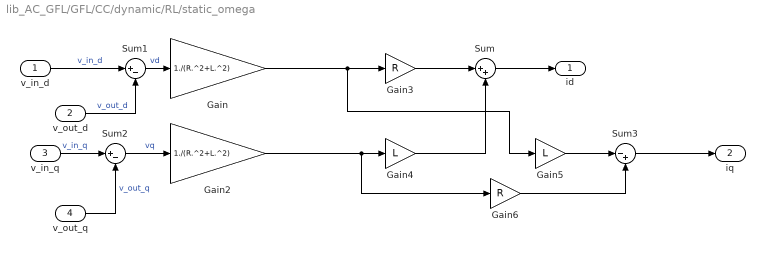
== system lib_AC_GFL/GFL/CC/dynamic/RL/static_omega ==
  v_in_d : Inport
  v_out_d : Inport  Port=2
  v_in_q : Inport  Port=3
  v_out_q : Inport  Port=4
  Gain : Gain  Gain=1./(R.^2+L.^2)
  Gain2 : Gain  Gain=1./(R.^2+L.^2)
  Gain3 : Gain  Gain=R
  Gain4 : Gain  Gain=L
  Gain5 : Gain  Gain=L
  Gain6 : Gain  Gain=R
  Sum : Sum  Inputs=|++
  Sum1 : Sum  Inputs=|+-
  Sum2 : Sum  Inputs=|+-
  Sum3 : Sum  Inputs=|-+
  id : Outport
  iq : Outport  Port=2
  wires:
  v_in_q/1 -> Sum2/1  "v_in_q"
  v_in_d/1 -> Sum1/1  "v_in_d"
  v_out_q/1 -> Sum2/2  "v_out_q"
  v_out_d/1 -> Sum1/2  "v_out_d"
  Sum1/1 -> Gain/1  "vd"
  Sum2/1 -> Gain2/1  "vq"
  Gain/1 -> Gain5/1, Gain3/1
  Gain3/1 -> Sum/1
  Gain4/1 -> Sum/2
  Gain2/1 -> Gain6/1, Gain4/1
  Sum/1 -> id/1
  Gain5/1 -> Sum3/1
  Sum3/1 -> iq/1
  Gain6/1 -> Sum3/2

== system lib_AC_GFL/GFL/PC/LPF_d/Active/Impl ==
  In1 : Inport
  Gain : Gain  Gain=iTf
  I : Integrator  InitialCondition=op_GFL.PC_LPF_d_Active_Impl_I
  Sum4 : Sum  Inputs=|+-
  Out1 : Outport
  wires:
  I/1 -> Out1/1, Sum4/2
  In1/1 -> Sum4/1
  Sum4/1 -> Gain/1
  Gain/1 -> I/1

== system lib_AC_GFL/GFL/PC/LPF_q/Active/Impl ==
  In1 : Inport
  Gain : Gain  Gain=iTf
  I : Integrator  InitialCondition=op_GFL.PC_LPF_q_Active_Impl_I
  Sum4 : Sum  Inputs=|+-
  Out1 : Outport
  wires:
  Sum4/1 -> Gain/1
  In1/1 -> Sum4/1
  I/1 -> Out1/1, Sum4/2
  Gain/1 -> I/1
